simulink model "afe_dqctrl_param"  (R2026a)
settings: Solver=ode23tb  StopTime=param.sim.simlength  FixedStep=tc  MaxStep=param.glb_time.tc
values from neighbouring files (symbols this model uses):
  param = add_template_extras(param, options)    [init_model.m]
undefined symbols (not defined in the file or in its folder): magnitude
libraries: fl_lib x166, nesl_utility x91, igbt_simple_2th_lib x6, single_phase_transformer_lib x3, discrete_time_low_pass_filter x1, threephase_inductor_lib x1, dclink_for_two_levels x1, three_phase_pwm_modulator x1, three_phase_voltage_with_frt_emulator x1
(part 1 of 7)
settings Model: Creator=dbagn  LastModifiedBy=d.bagnara
settings SolverCC: NumberNewtonIterations=3.0  ZeroCrossControl=DisableAll  SolverResetMethod=Robust
settings SFSimCC: CustomCodeUndefinedFunction=ThrowError  DefaultCustomCodeDeterministicFunctions=All
settings SFSimCC: SimCustomHeaderCode=|
  | #include "rpi.h"
  | #include "rpi_simulink.h"
  | #include "bemf_obsv_load_est.h"
  | #include "bemf_obsv_load_est_simulink.h"
  | #include "dqpll_grid.h"
  | #include "dsmavgflt.h"
  | #include "bemf_obsv.h"
  | #include "bemf_obsv_simulink.h"
  | #include "mavgflt.h"
  | #include "mavgflt_simulink.h"
  | #include "mavgflts.h"
  | #include "mavgflts_simulink.h"
  | #include "sv_pwm_cm.h"
  | #include "dsmavgflt_simulink.h"
  | #include "linear_double_integrator_observer_simulink.h"
  | #include "sv_pwm_cm_simulink.h"
  | #include "dqvector_pi.h"
  | #include "dqpll_grid_simulink.h"
  | #include "first_harmonic_tracker.h"
  | #include "dqvector_pi_simulink.h"
  | #include "first_harmonic_tracker_simulink.h"
  | #include "dqpll_thyr.h"
  | #include "sv_pwm_simulink.h"
  | #include "sv_pwm.h"
  | #include "dqpll_thyr_simulink.h"
  | #include "linear_double_integrator_observer.h"
  | #include "math_f.h"
settings SFSimCC: SimUserSources=|
  | "rpi.c"
  | "rpi_simulink.c"
  | "mavgflt_simulink.c"
  | "mavgflt.c"
  | "mavgflts_simulink.c"
  | "mavgflts.c"
  | "dsmavgflt_simulink.c"
  | "dsmavgflt.c"
  | "bemf_obsv_simulink.c"
  | "bemf_obsv.c"
  | "bemf_obsv_load_est_simulink.c"
  | "bemf_obsv_load_est.c"
  | "dqvector_pi.c"
  | "dqvector_pi_simulink.c"
  | "sv_pwm_simulink.c"
  | "sv_pwm.c"
  | "first_harmonic_tracker_simulink.c"
  | "first_harmonic_tracker.c"
  | "dqpll_thyr_simulink.c"
  | "dqpll_thyr.c"
  | "dqpll_grid_simulink.c"
  | "dqpll_grid.c"
  | "linear_double_integrator_observer_simulink.c"
  | "linear_double_integrator_observer.c"
  | "sv_pwm_cm_simulink.c"
  | "sv_pwm_cm.c"
settings SFSimCC: SimUserIncludeDirs=|
  | include
  | src
settings SimscapeCC: SimscapeNominalValues="[{\"value\":\"1\",\"unit\":\"A\"},{\"value\":\"1\",\"unit\":\"bar\"},{\"value\":\"1\",\"unit\":\"cm^2\"},{\"value\":\"1\",\"unit\":\"cm^3/s\"},{\"value\":\"1\",\"unit\":\"kJ/kg\"},{\"value\":\"1\",\"unit\":\"kW\"},{\"value\":\"1\",\"unit\":\"l\"},{\"value\":\"1\",\"unit\":\"N\"},{\"value\":\"1\",\"unit\":\"N*m\"},{\"value\":\"1\",\"unit\":\"V\"}]"  SimscapeLogType=none  SimscapeLogDataHistory=5000.0

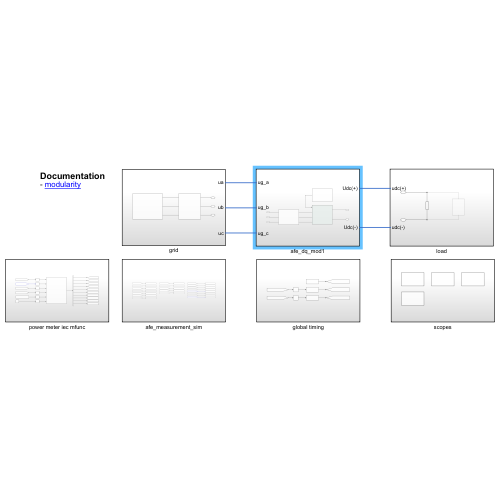
[thumbnail: Simulink's stored preview of the top-level diagram]
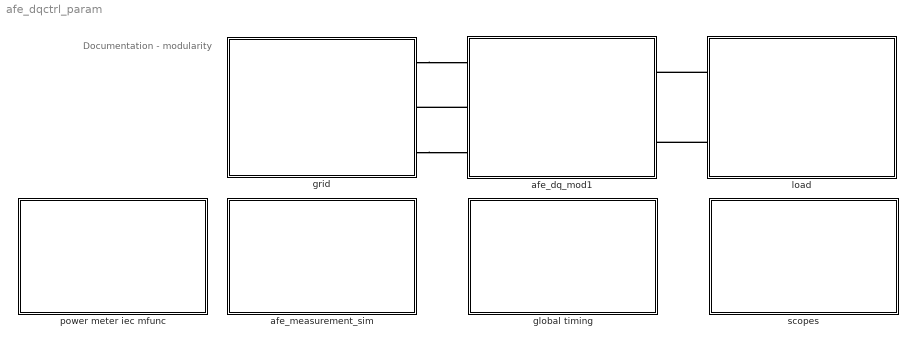
== system afe_dqctrl_param ==
  note: Documentation
      | - modularity
  afe_dq_mod1 : Subsystem
  afe_measurement_sim : Subsystem
  global timing : Subsystem
  grid : Subsystem
  load : Subsystem
  power meter iec mfunc : Subsystem
  scopes : Subsystem
  connections:
  grid/RConn1 -- afe_dq_mod1/LConn1
  grid/RConn3 -- afe_dq_mod1/LConn3
  afe_dq_mod1/LConn2 -- grid/RConn2
  load/LConn1 -- afe_dq_mod1/RConn1
  load/LConn2 -- afe_dq_mod1/RConn2

== system afe_dqctrl_param/afe_dq_mod1 ==
  AFE_control : Subsystem
  LCL_filter : Subsystem
  afe : Subsystem
  ug_a : PMIOPort  Side=Left
  ug_b : PMIOPort  Port=2  Side=Left
  ug_c : PMIOPort  Port=3  Side=Left
  Udc(+) : PMIOPort  Port=4  Side=Right
  Udc(-) : PMIOPort  Port=5  Side=Right
  wires:
  AFE_control/1(dabc_out) -> afe/1(dabc)
  connections:
  Udc(-)/RConn1 -- afe/RConn2
  Udc(+)/RConn1 -- afe/RConn1
  LCL_filter/LConn1 -- afe/LConn1
  LCL_filter/LConn2 -- afe/LConn2
  LCL_filter/LConn3 -- afe/LConn3
  ug_a/RConn1 -- LCL_filter/RConn1
  ug_b/RConn1 -- LCL_filter/RConn2
  ug_c/RConn1 -- LCL_filter/RConn3

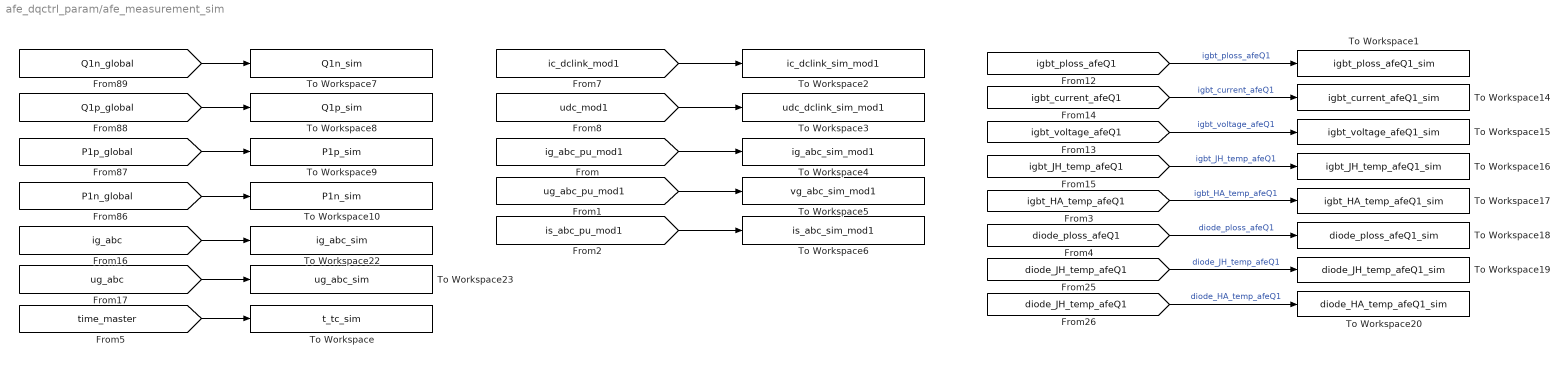
== system afe_dqctrl_param/afe_measurement_sim ==
  To Workspace : ToWorkspace  VariableName=t_tc_sim  SampleTime=param.glb_time.tc
      settings: MaxDataPoints=param.glb_time.Nc
  To Workspace1 : ToWorkspace  VariableName=igbt_ploss_afeQ1_sim  SampleTime=param.glb_time.tc
      settings: MaxDataPoints=param.glb_time.Nc
  To Workspace10 : ToWorkspace  VariableName=P1n_sim  SampleTime=param.glb_time.ts_afe
      settings: MaxDataPoints=param.glb_time.Ns_afe
  To Workspace14 : ToWorkspace  VariableName=igbt_current_afeQ1_sim  SampleTime=param.glb_time.tc
      settings: MaxDataPoints=param.glb_time.Nc
  To Workspace15 : ToWorkspace  VariableName=igbt_voltage_afeQ1_sim  SampleTime=param.glb_time.tc
      settings: MaxDataPoints=param.glb_time.Nc
  To Workspace16 : ToWorkspace  VariableName=igbt_JH_temp_afeQ1_sim  SampleTime=param.glb_time.tc
      settings: MaxDataPoints=param.glb_time.Nc
  To Workspace17 : ToWorkspace  VariableName=igbt_HA_temp_afeQ1_sim  SampleTime=param.glb_time.tc
      settings: MaxDataPoints=param.glb_time.Nc
  To Workspace18 : ToWorkspace  VariableName=diode_ploss_afeQ1_sim  SampleTime=param.glb_time.tc
      settings: MaxDataPoints=param.glb_time.Nc
  To Workspace19 : ToWorkspace  VariableName=diode_JH_temp_afeQ1_sim  SampleTime=param.glb_time.tc
      settings: MaxDataPoints=param.glb_time.Nc
  To Workspace2 : ToWorkspace  VariableName=ic_dclink_sim_mod1  SampleTime=param.glb_time.tc
      settings: MaxDataPoints=param.glb_time.Nc
  To Workspace20 : ToWorkspace  VariableName=diode_HA_temp_afeQ1_sim  SampleTime=param.glb_time.tc
      settings: MaxDataPoints=param.glb_time.Nc
  To Workspace22 : ToWorkspace  VariableName=ig_abc_sim  SampleTime=param.glb_time.tc
      settings: MaxDataPoints=param.glb_time.Nc
  To Workspace23 : ToWorkspace  VariableName=ug_abc_sim  SampleTime=param.glb_time.tc
      settings: MaxDataPoints=param.glb_time.Nc
  To Workspace3 : ToWorkspace  VariableName=udc_dclink_sim_mod1  SampleTime=param.glb_time.tc
      settings: MaxDataPoints=param.glb_time.Nc
  To Workspace4 : ToWorkspace  VariableName=ig_abc_sim_mod1  SampleTime=param.glb_time.tc
      settings: MaxDataPoints=param.glb_time.Nc
  To Workspace5 : ToWorkspace  VariableName=vg_abc_sim_mod1  SampleTime=param.glb_time.tc
      settings: MaxDataPoints=param.glb_time.Nc
  To Workspace6 : ToWorkspace  VariableName=is_abc_sim_mod1  SampleTime=param.glb_time.tc
      settings: MaxDataPoints=param.glb_time.Nc
  To Workspace7 : ToWorkspace  VariableName=Q1n_sim  SampleTime=param.glb_time.ts_afe
      settings: MaxDataPoints=param.glb_time.Ns_afe
  To Workspace8 : ToWorkspace  VariableName=Q1p_sim  SampleTime=param.glb_time.ts_afe
      settings: MaxDataPoints=param.glb_time.Ns_afe
  To Workspace9 : ToWorkspace  VariableName=P1p_sim  SampleTime=param.glb_time.ts_afe
      settings: MaxDataPoints=param.glb_time.Ns_afe
  wires:
  [time_master] -> To Workspace/1
  [Q1n_global] -> To Workspace7/1
  [Q1p_global] -> To Workspace8/1
  [P1p_global] -> To Workspace9/1
  [P1n_global] -> To Workspace10/1
  [ug_abc] -> To Workspace23/1
  [ig_abc] -> To Workspace22/1
  [ug_abc_pu_mod1] -> To Workspace5/1
  [ig_abc_pu_mod1] -> To Workspace4/1
  [udc_mod1] -> To Workspace3/1
  [ic_dclink_mod1] -> To Workspace2/1
  [is_abc_pu_mod1] -> To Workspace6/1
  [igbt_voltage_afeQ1] -> To Workspace15/1  "igbt_voltage_afeQ1"
  [igbt_HA_temp_afeQ1] -> To Workspace17/1  "igbt_HA_temp_afeQ1"
  [diode_ploss_afeQ1] -> To Workspace18/1  "diode_ploss_afeQ1"
  [diode_JH_temp_afeQ1] -> To Workspace19/1  "diode_JH_temp_afeQ1"
  [igbt_ploss_afeQ1] -> To Workspace1/1  "igbt_ploss_afeQ1"
  [diode_JH_temp_afeQ1] -> To Workspace20/1  "diode_HA_temp_afeQ1"
  [igbt_current_afeQ1] -> To Workspace14/1  "igbt_current_afeQ1"
  [igbt_JH_temp_afeQ1] -> To Workspace16/1  "igbt_JH_temp_afeQ1"

== system afe_dqctrl_param/global timing ==
  Unit Delay : UnitDelay  SampleTime=param.glb_time.tc
  Unit Delay1 : UnitDelay  SampleTime=param.glb_time.tc
  time_afe1 : Subsystem  mask{k=param.afe.behav.time_gain_module_1}
      mask prompts: k "Time Gain"
      mask Display:
      | disp('time-gen');
      | port_label('input', 1, 'crt');
      | port_label('output', 1, 'tout');
  time_afe3 : Subsystem  mask{k=1}
      mask prompts: k "Time Gain"
      mask Display:
      | disp('time-gen');
      | port_label('output', 1, 'tout');
  time_inv1 : Subsystem  mask{k=param.inv.behav.time_gain_module_2}
      mask prompts: k "Time Gain"
      mask Display:
      | disp('time-gen');
      | port_label('input', 1, 'crt');
      | port_label('output', 1, 'tout');
  tag scope: time_afe_module_1=global, time_inv_module_1=global, time_master=global
  wires:
  time_afe1/1(Out1) -> [time_afe_module_1]
  time_inv1/1(Out1) -> [time_inv_module_1]
  time_afe3/1(Out1) -> [time_master]
  [local_time_corr_afe1] -> Unit Delay/1
  Unit Delay/1 -> time_afe1/1(correction_time)
  [local_time_corr_inv1] -> Unit Delay1/1
  Unit Delay1/1 -> time_inv1/1(correction_time)

== system afe_dqctrl_param/grid ==
  grid_emulator : Subsystem
  threephase_vi_measures : Subsystem
  ua : PMIOPort  Side=Right
  ub : PMIOPort  Port=2  Side=Right
  uc : PMIOPort  Port=3  Side=Right
  connections:
  threephase_vi_measures/LConn3 -- grid_emulator/RConn3
  threephase_vi_measures/LConn1 -- grid_emulator/RConn1
  threephase_vi_measures/RConn2 -- ub/RConn1
  threephase_vi_measures/LConn2 -- grid_emulator/RConn2
  threephase_vi_measures/RConn1 -- ua/RConn1
  threephase_vi_measures/RConn3 -- uc/RConn1

== system afe_dqctrl_param/load ==
  load : fl_lib/Electrical/Electrical Elements/Resistor  R=1070^2/275e3 Ohm  i_specify=off  i_priority=None  i=0 A  i_nominal_specify=off  i_nominal_value=1  i_nominal_unit=A  v_specify=off  v_priority=None  v=0 V  v_nominal_specify=off  v_nominal_value=1  v_nominal_unit=V
  load_current_source : Subsystem  Commented=on
  udc(+) : PMIOPort  Side=Left
  udc(-) : PMIOPort  Port=2  Side=Left
  connections:
  load/RConn1 -- udc(-)/RConn1 -- load_current_source/RConn1
  udc(+)/RConn1 -- load_current_source/LConn1 -- load/LConn1

== system afe_dqctrl_param/power meter iec mfunc ==
  Bus Selector : BusSelector  OutputSignals=Q1p,Q1n,P1n,P1p,U1n,U1p,i_act_1n,i_react_1n,i_act_1p,i_react_1p
  Constant : Constant  Value=param.glb_time.ts_afe
  Step : Step  Time=0.025  InitialValue=1  FinalValue=0  SampleTime=0
  To Workspace1 : ToWorkspace  VariableName=i_react_1n  SampleTime=param.glb_time.ts_afe
      settings: MaxDataPoints=param.glb_time.Ns_afe
  To Workspace2 : ToWorkspace  VariableName=i_react_1p  SampleTime=param.glb_time.ts_afe
      settings: MaxDataPoints=param.glb_time.Ns_afe
  To Workspace3 : ToWorkspace  VariableName=i_act_1n  SampleTime=param.glb_time.ts_afe
      settings: MaxDataPoints=param.glb_time.Ns_afe
  To Workspace4 : ToWorkspace  VariableName=i_act_1p  SampleTime=param.glb_time.ts_afe
      settings: MaxDataPoints=param.glb_time.Ns_afe
  To Workspace5 : ToWorkspace  VariableName=u1p  SampleTime=param.glb_time.ts_afe
      settings: MaxDataPoints=param.glb_time.Ns_afe
  To Workspace6 : ToWorkspace  VariableName=u1n  SampleTime=param.glb_time.ts_afe
      settings: MaxDataPoints=param.glb_time.Ns_afe
  Zero-Order Hold{,1..5} (6 alike) : ZeroOrderHold  SampleTime=param.glb_time.ts_afe
  three_phase_power_meter_iec : MATLAB Function  TreatAsAtomicUnit=on  SystemSampleTime=param.glb_time.ts_afe
  tag scope: P1n_global=global, P1p_global=global, Q1n_global=global, Q1p_global=global
  wires:
  Bus Selector/6 -> To Workspace5/1  "<U1p>"
  Bus Selector/8 -> To Workspace1/1  "<i_react_1n>"
  Bus Selector/10 -> To Workspace2/1  "<i_react_1p>"
  Bus Selector/5 -> To Workspace6/1  "<U1n>"
  Bus Selector/4 -> [P1p_global]  "<P1p>"
  Bus Selector/2 -> [Q1n_global]  "<Q1n>"
  Bus Selector/1 -> [Q1p_global]  "<Q1p>"
  Bus Selector/7 -> To Workspace3/1  "<i_act_1n>"
  Bus Selector/9 -> To Workspace4/1  "<i_act_1p>"
  Bus Selector/3 -> [P1n_global]  "<P1n>"
  three_phase_power_meter_iec/1(m) -> Bus Selector/1
  Zero-Order Hold/1 -> three_phase_power_meter_iec/1(phase)
  Zero-Order Hold2/1 -> three_phase_power_meter_iec/3(i_abc)
  [gamma_grid_emulator] -> Zero-Order Hold/1
  Step/1 -> Zero-Order Hold5/1
  Zero-Order Hold3/1 -> three_phase_power_meter_iec/4(omega)
  Zero-Order Hold4/1 -> three_phase_power_meter_iec/5(ts)
  [ug_abc] -> Zero-Order Hold1/1
  Zero-Order Hold5/1 -> three_phase_power_meter_iec/6(enable_time)
  [ig_abc] -> Zero-Order Hold2/1
  [omega_grid_emulator] -> Zero-Order Hold3/1
  Constant/1 -> Zero-Order Hold4/1
  Zero-Order Hold1/1 -> three_phase_power_meter_iec/2(u_abc)

== system afe_dqctrl_param/scopes ==
  cable_effects : Subsystem
  grid_afe_side : Subsystem
  igbt_power_losses : Subsystem
  mosfet_power_losses : Subsystem  Commented=on

== system afe_dqctrl_param/afe_dq_mod1/AFE_control ==
  To Workspace : ToWorkspace  VariableName=afe_ctrl_data_output_mod1  SampleTime=param.glb_time.ts_afe
      settings: MaxDataPoints=param.glb_time.Ns_afe
  afe_control : Subsystem
  dabc_out : Outport
  tag scope: local_time_corr_afe1=global
  wires:
  [TRGO_afe_module_1] -> afe_control/Trigger
  [ug_abc_pu_mod1] -> afe_control/1(ug_abc_pu)
  [is_abc_pu_mod1] -> afe_control/4(is_abc_pu)
  [vdc_pu_afe_mod1] -> afe_control/2(udc_pu)
  afe_control/1(duvw) -> dabc_out/1
  [ig_abc_pu_mod1] -> afe_control/3(ig_abc_pu)
  [time_afe_module_1] -> afe_control/5(local_time)
  [time_master] -> afe_control/6(master_time)
  [gamma_grid_emulator] -> afe_control/7(grid_phase)
  afe_control/3(m_data) -> To Workspace/1
  afe_control/2(AFE1_local_time_corr) -> [local_time_corr_afe1]

== system afe_dqctrl_param/afe_dq_mod1/LCL_filter ==
  CFu1 : fl_lib/Electrical/Electrical Elements/Capacitor  c=param.afe.hw.CFu F  r=param.afe.hw.RCFu Ohm  g=0 1/Ohm  i_specify=off  i_priority=None  i=0 A  i_nominal_specify=off  i_nominal_value=1  i_nominal_unit=A  v_specify=off  v_priority=None  v=0 V  v_nominal_specify=off  v_nominal_value=1  v_nominal_unit=V  vc_specify=off  vc_priority=High  vc=0 V  vc_nominal_specify=off  vc_nominal_value=1  vc_nominal_unit=V
  CFu2 : fl_lib/Electrical/Electrical Elements/Capacitor  c=param.afe.hw.CFu F  r=param.afe.hw.RCFu Ohm  g=0 1/Ohm  i_specify=off  i_priority=None  i=0 A  i_nominal_specify=off  i_nominal_value=1  i_nominal_unit=A  v_specify=off  v_priority=None  v=0 V  v_nominal_specify=off  v_nominal_value=1  v_nominal_unit=V  vc_specify=off  vc_priority=High  vc=0 V  vc_nominal_specify=off  vc_nominal_value=1  vc_nominal_unit=V
  CFu3 : fl_lib/Electrical/Electrical Elements/Capacitor  c=param.afe.hw.CFu F  r=param.afe.hw.RCFu Ohm  g=0 1/Ohm  i_specify=off  i_priority=None  i=0 A  i_nominal_specify=off  i_nominal_value=1  i_nominal_unit=A  v_specify=off  v_priority=None  v=0 V  v_nominal_specify=off  v_nominal_value=1  v_nominal_unit=V  vc_specify=off  vc_priority=High  vc=0 V  vc_nominal_specify=off  vc_nominal_value=1  vc_nominal_unit=V
  Inductor : fl_lib/Electrical/Electrical Elements/Inductor  l=1e-6 H  r=0 Ohm  g=1e-9 1/Ohm  i_specify=on  i_priority=High  i=0 A  i_nominal_specify=off  i_nominal_value=1  i_nominal_unit=A  v_specify=off  v_priority=None  v=0 V  v_nominal_specify=off  v_nominal_value=1  v_nominal_unit=V  i_L_specify=off  i_L_priority=High  i_L=0 A  i_L_nominal_specify=off  i_L_nominal_value=1  i_L_nominal_unit=A
  Inductor1 : fl_lib/Electrical/Electrical Elements/Inductor  l=1e-6 H  r=0 Ohm  g=1e-9 1/Ohm  i_specify=on  i_priority=High  i=0 A  i_nominal_specify=off  i_nominal_value=1  i_nominal_unit=A  v_specify=off  v_priority=None  v=0 V  v_nominal_specify=off  v_nominal_value=1  v_nominal_unit=V  i_L_specify=off  i_L_priority=High  i_L=0 A  i_L_nominal_specify=off  i_L_nominal_value=1  i_L_nominal_unit=A
  Inductor2 : fl_lib/Electrical/Electrical Elements/Inductor  l=1e-6 H  r=0 Ohm  g=1e-9 1/Ohm  i_specify=on  i_priority=High  i=0 A  i_nominal_specify=off  i_nominal_value=1  i_nominal_unit=A  v_specify=off  v_priority=None  v=0 V  v_nominal_specify=off  v_nominal_value=1  v_nominal_unit=V  i_L_specify=off  i_L_priority=High  i_L=0 A  i_L_nominal_specify=off  i_L_nominal_value=1  i_L_nominal_unit=A
  threephase inductor : threephase_inductor_lib/threephase inductor  Lp=param.afe.hw.LFu H  L0=param.afe.hw.LFu_cm H  Rp=param.afe.hw.RLFu Ohm  R0=param.afe.hw.RLFu_cm Ohm  Lls=5e-6 H  uu_1_specify=off  uu_1_priority=None  uu_1=0 V  uu_1_nominal_specify=off  uu_1_nominal_value=1  uu_1_nominal_unit=V  uv_1_specify=off  uv_1_priority=None  uv_1=0 V  uv_1_nominal_specify=off  uv_1_nominal_value=1  uv_1_nominal_unit=V  uw_1_specify=off  uw_1_priority=None  uw_1=0 V  uw_1_nominal_specify=off  uw_1_nominal_value=1  uw_1_nominal_unit=V  uu_2_specify=off  uu_2_priority=None  uu_2=0 V  uu_2_nominal_specify=off  uu_2_nominal_value=1  uu_2_nominal_unit=V  uv_2_specify=off  uv_2_priority=None  uv_2=0 V  uv_2_nominal_specify=off  uv_2_nominal_value=1  uv_2_nominal_unit=V  uw_2_specify=off  uw_2_priority=None  uw_2=0 V  uw_2_nominal_specify=off  uw_2_nominal_value=1  uw_2_nominal_unit=V  iu_specify=off  iu_priority=High  iu=0 A  iu_nominal_specify=off  iu_nominal_value=1  iu_nominal_unit=A  iv_specify=off  iv_priority=High  iv=0 A  iv_nominal_specify=off  iv_nominal_value=1  iv_nominal_unit=A  iw_specify=off  iw_priority=High  iw=0 A  iw_nominal_specify=off  iw_nominal_value=1  iw_nominal_unit=A
  threephase_vi_measures_stack : Subsystem
  threephase_vi_measures_stack1 : Subsystem
  us_a : PMIOPort  Side=Left
  ug_a : PMIOPort  Port=2  Side=Right
  us_b : PMIOPort  Port=3  Side=Left
  ug_b : PMIOPort  Port=4  Side=Right
  us_c : PMIOPort  Port=5  Side=Left
  ug_c : PMIOPort  Port=6  Side=Right
  connections:
  CFu1/RConn1 -- CFu3/RConn1 -- CFu2/RConn1
  Inductor/RConn1 -- threephase_vi_measures_stack1/LConn1 -- CFu1/LConn1
  Inductor2/RConn1 -- CFu3/LConn1 -- threephase_vi_measures_stack1/LConn3
  Inductor1/RConn1 -- CFu2/LConn1 -- threephase_vi_measures_stack1/LConn2
  threephase_vi_measures_stack/LConn1 -- us_a/RConn1
  threephase_vi_measures_stack/LConn2 -- us_b/RConn1
  threephase_vi_measures_stack/LConn3 -- us_c/RConn1
  threephase_vi_measures_stack/RConn1 -- threephase inductor/LConn1
  threephase_vi_measures_stack/RConn2 -- threephase inductor/LConn2
  threephase_vi_measures_stack/RConn3 -- threephase inductor/LConn3
  threephase inductor/RConn1 -- Inductor/LConn1
  Inductor1/LConn1 -- threephase inductor/RConn2
  Inductor2/LConn1 -- threephase inductor/RConn3
  ug_a/RConn1 -- threephase_vi_measures_stack1/RConn1
  ug_b/RConn1 -- threephase_vi_measures_stack1/RConn2
  ug_c/RConn1 -- threephase_vi_measures_stack1/RConn3

== system afe_dqctrl_param/afe_dq_mod1/afe ==
  dabc : Inport
  Bus Selector : BusSelector  OutputSignals=vdc_pu
  Bus Selector1 : BusSelector  OutputSignals=udc,udc_p_gnd,udc_centertap_gnd,udc_n_gnd  OutputAsBus=on
  Bus Selector2 : BusSelector  OutputSignals=udc
  Bus Selector3 : BusSelector  OutputSignals=Cdc1_current
  dclink1 : dclink_for_two_levels/dclink  Cdc=param.afe.hw.CFi  Rudc_measure=1e6  Vdc_scale=param.afe.hw.udc_nom
  sv_pwm : Subsystem
  three_phase_inverter_with_igbt_simple_2th : Subsystem
  us_a : PMIOPort  Side=Left
  us_b : PMIOPort  Port=2  Side=Left
  us_c : PMIOPort  Port=3  Side=Left
  Udc(+) : PMIOPort  Port=4  Side=Right
  Udc(-) : PMIOPort  Port=5  Side=Right
  tag scope: all_voltages_about_dclink=global, ic_dclink_mod1=global, udc_mod1=global, vdc_pu_afe_mod1=global, vdc_pu_inv_mod1=global
  wires:
  dabc/1 -> sv_pwm/1(duties_uvw)
  sv_pwm/1(gate_cmds) -> three_phase_inverter_with_igbt_simple_2th/1(gate_commands)
  dclink1/1 -> Bus Selector1/1, Bus Selector2/1, Bus Selector3/1, Bus Selector/1
  Bus Selector1/1 -> [all_voltages_about_dclink]
  Bus Selector/1 -> [vdc_pu_afe_mod1], [vdc_pu_inv_mod1]  "<vdc_pu>"
  Bus Selector2/1 -> [udc_mod1]  "<udc>"
  Bus Selector3/1 -> [ic_dclink_mod1]  "<Cdc1_current>"
  connections:
  three_phase_inverter_with_igbt_simple_2th/RConn2 -- us_b/RConn1
  dclink1/RConn1 -- Udc(+)/RConn1
  dclink1/RConn2 -- Udc(-)/RConn1
  three_phase_inverter_with_igbt_simple_2th/RConn1 -- us_a/RConn1
  three_phase_inverter_with_igbt_simple_2th/RConn3 -- us_c/RConn1
  dclink1/LConn2 -- three_phase_inverter_with_igbt_simple_2th/LConn2
  dclink1/LConn1 -- three_phase_inverter_with_igbt_simple_2th/LConn1

== system afe_dqctrl_param/global timing/time_afe1 ==
  correction_time : Inport
  Constant : Constant
  Gain : Gain  Gain=k
  Product : Product
  Sum : Sum  Inputs=|++
  time_1 : Clock
  Out1 : Outport
  wires:
  time_1/1 -> Gain/1
  Gain/1 -> Product/1
  Product/1 -> Out1/1
  correction_time/1 -> Sum/1
  Sum/1 -> Product/2
  Constant/1 -> Sum/2

== system afe_dqctrl_param/global timing/time_afe3 ==
  Gain : Gain  Gain=k
  time_1 : Clock
  Out1 : Outport
  wires:
  Gain/1 -> Out1/1
  time_1/1 -> Gain/1

== system afe_dqctrl_param/global timing/time_inv1 ==
  correction_time : Inport
  Constant : Constant
  Gain : Gain  Gain=k
  Product : Product
  Sum : Sum  Inputs=|++
  time_1 : Clock
  Out1 : Outport
  wires:
  time_1/1 -> Gain/1
  Gain/1 -> Product/1
  Product/1 -> Out1/1
  correction_time/1 -> Sum/1
  Constant/1 -> Sum/2
  Sum/1 -> Product/2

== system afe_dqctrl_param/grid/grid_emulator ==
  3ph_Dyg : Subsystem
  Bus Selector : BusSelector  OutputSignals=ua_grid_emu,ub_grid_emu,uc_grid_emu
  Bus Selector1 : BusSelector  OutputSignals=gamma_grid_emulator,omega_grid_emulator
  Controlled Voltage Source : fl_lib/Electrical/Electrical Sources/Controlled Voltage Source
  Controlled Voltage Source1 : fl_lib/Electrical/Electrical Sources/Controlled Voltage Source
  Controlled Voltage Source2 : fl_lib/Electrical/Electrical Sources/Controlled Voltage Source
  Electrical Reference : fl_lib/Electrical/Electrical Elements/Electrical Reference
  Simulink-PS Converter : nesl_utility/Simulink-PS Converter  PhysicalDomain=network_engine_domain  SubClassName=ps_input  LeftPortType=input  RightPortType=output  PseudoPeriodic=off  Frequencies=[]  NoiseDistribution=none  NoiseParameters=[]  Unit=V  AffineConversion=on  FilteringAndDerivatives=provide  SimscapeFilterOrder=1  InputFilterTimeConstant=0.001  UdotUserProvided=0
  Simulink-PS Converter1 : nesl_utility/Simulink-PS Converter  PhysicalDomain=network_engine_domain  SubClassName=ps_input  LeftPortType=input  RightPortType=output  PseudoPeriodic=off  Frequencies=[]  NoiseDistribution=none  NoiseParameters=[]  Unit=V  AffineConversion=on  FilteringAndDerivatives=provide  SimscapeFilterOrder=1  InputFilterTimeConstant=0.001  UdotUserProvided=0
  Simulink-PS Converter2 : nesl_utility/Simulink-PS Converter  PhysicalDomain=network_engine_domain  SubClassName=ps_input  LeftPortType=input  RightPortType=output  PseudoPeriodic=off  Frequencies=[]  NoiseDistribution=none  NoiseParameters=[]  Unit=V  AffineConversion=on  FilteringAndDerivatives=provide  SimscapeFilterOrder=1  InputFilterTimeConstant=0.001  UdotUserProvided=0
  Solver Configuration : nesl_utility/Solver Configuration  PhysicalDomain=network_engine_domain  SubClassName=solver  LeftPortType=input  RightPortType=generic  Tones=[]  Harmonics=[]  SimulateNoise=off  Profile=off  UseLocalSampling=off  EnableSwitchedLinearOptims=on  FrequencyDomain=off  UseCCode=off  RelTol=0.001  AbsTol=0.001  MinStep=1e-09  ToWorkspace=off  RevertToSquareIcSolve=off  NumHomotopyIterations=100  PhasorMode=off  PhasorModeNumHarmonics=1  ConsistencySolver=NEWTON_FTOL  CanonicalOrdering=UNORDERED  OptimizeIntermediates=UNOPTIMIZED  IndexReductionMethod=DerivativeReplacement  DoDC=on  ResidualTolerance=1e-3  ConsistencyTolSource=GLOBAL  ConsistencyAbsTol=0.001  ConsistencyRelTol=0.001  ConsistencyTolFactor=0.001  UseLocalSolver=on  LocalSolverChoice=NE_BACKWARD_EULER_ADVANCER  ResolveIndetEquations=on  FunctionEvalNumThread=1  LocalSolverSampleTime=param.glb_time.tc  DoFixedCost=on  MaxNonlinIter=param.sim.nonlinear_iterations  MaxModeIter=2  ComputeImpulses=off  ImpulseIterations=2  LinearAlgebra=auto  LinearAlgebraNumThread=0  EquationFormulation=NE_TIME_EF  DelaysMemoryBudget=1024  AutomaticFiltering=on  FilteringTimeConstant=0.001  PartitionStorageMethod=AS_NEEDED  PartitionMemoryBudget=1024  PartitionMethod=ROBUST  MultibodyUseLocalSolver=off  MultibodyLocalSolverChoice=ODE1  MultibodyLocalSolverSampleTime=0.001
  three_phase_voltage_source_with_frt_emulator : three_phase_voltage_with_frt_emulator/three_phase_voltage_source_with_frt_emulator  nominal_frequency_m=param.grid.emu.fgrid_nom  nominal_voltage_m=param.grid.emu.us_primary_nom  Vemu_ref_norm_m=param.grid.emu.Vemu_ref_norm  vp_xi_pu_m=param.grid.emu.up_xi_pu_ref  vp_eta_pu_m=param.grid.emu.up_eta_pu_ref  vn_xi_pu_m=param.grid.emu.un_xi_pu_ref  vn_eta_pu_m=param.grid.emu.un_eta_pu_ref  Am=param.ctrl.filters.afe.SOF_50Hz.ss_c.A  Bm=param.ctrl.filters.afe.SOF_50Hz.ss_c.B  Cm=param.ctrl.filters.afe.SOF_50Hz.ss_c.C  enable_frt_1_m=param.frt.data.enable_frt_1  enable_frt_2_m=param.frt.data.enable_frt_2  start_time_LVRT_m=param.frt.data.start_time_LVRT  end_time_LVRT_m=param.frt.data.end_time_LVRT  deepPOSxi_m=param.frt.data.deepPOSxi  deepPOSeta_m=param.frt.data.deepPOSeta  deepNEGxi_m=param.frt.data.deepNEGxi  deepNEGeta_m=param.frt.data.deepNEGeta  Amplitude_U_m=param.frt.data.Amplitude_U  Amplitude_V_m=param.frt.data.Amplitude_V  Amplitude_W_m=param.frt.data.Amplitude_W  t_ramp_m=param.frt.data.t_ramp  Phase_shift_m=param.frt.data.Phase_shift
  threephase_vi_measures : Subsystem
  u1 : PMIOPort  Side=Right
  u2 : PMIOPort  Port=2  Side=Right
  u3 : PMIOPort  Port=3  Side=Right
  tag scope: gamma_grid_emulator=global, omega_grid_emulator=global
  wires:
  Bus Selector1/2 -> [omega_grid_emulator]  "<omega_grid_emulator>"
  Bus Selector1/1 -> [gamma_grid_emulator]  "<gamma_grid_emulator>"
  Bus Selector/2 -> Simulink-PS Converter1/1  "<ub_grid_emu>"
  Bus Selector/3 -> Simulink-PS Converter2/1  "<uc_grid_emu>"
  three_phase_voltage_source_with_frt_emulator/1 -> Bus Selector1/1, Bus Selector/1
  Bus Selector/1 -> Simulink-PS Converter/1  "<ua_grid_emu>"
  connections:
  Simulink-PS Converter/RConn1 -- Controlled Voltage Source/RConn1
  Simulink-PS Converter1/RConn1 -- Controlled Voltage Source1/RConn1
  Simulink-PS Converter2/RConn1 -- Controlled Voltage Source2/RConn1
  Electrical Reference/LConn1 -- Controlled Voltage Source/RConn2 -- Controlled Voltage Source1/RConn2 -- Controlled Voltage Source2/RConn2 -- Solver Configuration/RConn1
  3ph_Dyg/RConn1 -- u1/RConn1
  3ph_Dyg/RConn2 -- u2/RConn1
  3ph_Dyg/RConn3 -- u3/RConn1
  3ph_Dyg/LConn1 -- threephase_vi_measures/RConn1
  3ph_Dyg/LConn2 -- threephase_vi_measures/RConn2
  3ph_Dyg/LConn3 -- threephase_vi_measures/RConn3
  Controlled Voltage Source/LConn1 -- threephase_vi_measures/LConn1
  Controlled Voltage Source1/LConn1 -- threephase_vi_measures/LConn2
  Controlled Voltage Source2/LConn1 -- threephase_vi_measures/LConn3

== system afe_dqctrl_param/grid/threephase_vi_measures ==
  Bus Creator : BusCreator  Inputs=6
  Current Sensor : fl_lib/Electrical/Electrical Sensors/Current Sensor
  Current Sensor1 : fl_lib/Electrical/Electrical Sensors/Current Sensor
  Current Sensor2 : fl_lib/Electrical/Electrical Sensors/Current Sensor
  Electrical Reference1 : fl_lib/Electrical/Electrical Elements/Electrical Reference
  Selector : Selector  InputPortWidth=6  IndexOptions=Index vector (dialog)  Indices=[1 2 3]  OutputSizes=1
  Selector1 : Selector  InputPortWidth=6  IndexOptions=Index vector (dialog)  Indices=[4 5 6]  OutputSizes=1
  Voltage Sensor : fl_lib/Electrical/Electrical Sensors/Voltage Sensor
  Voltage Sensor1 : fl_lib/Electrical/Electrical Sensors/Voltage Sensor
  Voltage Sensor2 : fl_lib/Electrical/Electrical Sensors/Voltage Sensor
  ia_grid : nesl_utility/PS-Simulink Converter  PhysicalDomain=network_engine_domain  SubClassName=ps_output  LeftPortType=input  RightPortType=output  PseudoPeriodic=off  Frequencies=[]  VectorFormat=1-D array  Unit=A  AffineConversion=off
  ib_grid : nesl_utility/PS-Simulink Converter  PhysicalDomain=network_engine_domain  SubClassName=ps_output  LeftPortType=input  RightPortType=output  PseudoPeriodic=off  Frequencies=[]  VectorFormat=1-D array  Unit=A  AffineConversion=off
  ic_grid : nesl_utility/PS-Simulink Converter  PhysicalDomain=network_engine_domain  SubClassName=ps_output  LeftPortType=input  RightPortType=output  PseudoPeriodic=off  Frequencies=[]  VectorFormat=1-D array  Unit=A  AffineConversion=off
  ig_abc/ug_abc : Scope  NumInputPorts=2
      settings: SampleTime=param.glb_time.tc  ActiveDisplayYMinimum=-728.92703752654245  ActiveDisplayYMaximum=734.90808013997  DataLoggingVariableName=ScopeData2
  ua_grid : nesl_utility/PS-Simulink Converter  PhysicalDomain=network_engine_domain  SubClassName=ps_output  LeftPortType=input  RightPortType=output  PseudoPeriodic=off  Frequencies=[]  VectorFormat=1-D array  Unit=V  AffineConversion=off
  ub_grid : nesl_utility/PS-Simulink Converter  PhysicalDomain=network_engine_domain  SubClassName=ps_output  LeftPortType=input  RightPortType=output  PseudoPeriodic=off  Frequencies=[]  VectorFormat=1-D array  Unit=V  AffineConversion=off
  uc_grid : nesl_utility/PS-Simulink Converter  PhysicalDomain=network_engine_domain  SubClassName=ps_output  LeftPortType=input  RightPortType=output  PseudoPeriodic=off  Frequencies=[]  VectorFormat=1-D array  Unit=V  AffineConversion=off
  Ua : PMIOPort  Side=Left
  ua : PMIOPort  Port=2  Side=Right
  Ub : PMIOPort  Port=3  Side=Left
  ub : PMIOPort  Port=4  Side=Right
  Uc : PMIOPort  Port=5  Side=Left
  uc : PMIOPort  Port=6  Side=Right
  tag scope: ig_abc=global, ug_abc=global
  wires:
  Bus Creator/1 -> Selector1/1, Selector/1  "vi_data"
  Selector/1 -> [ug_abc]
  ib_grid/1 -> Bus Creator/5  "ib"
  ia_grid/1 -> Bus Creator/4  "ia"
  ic_grid/1 -> Bus Creator/6  "ic"
  ua_grid/1 -> Bus Creator/1  "ua"
  ub_grid/1 -> Bus Creator/2  "ub"
  uc_grid/1 -> Bus Creator/3  "uc"
  Selector1/1 -> [ig_abc]
  [ug_abc] -> ig_abc/ug_abc/2  "ug_abc(line)"
  [ig_abc] -> ig_abc/ug_abc/1  "ig_abc(line)"
  connections:
  Current Sensor1/LConn1 -- Ub/RConn1 -- Voltage Sensor1/LConn1
  Electrical Reference1/LConn1 -- Voltage Sensor/RConn2 -- Voltage Sensor2/RConn2 -- Voltage Sensor1/RConn2
  Voltage Sensor/RConn1 -- ua_grid/LConn1
  Current Sensor/RConn2 -- ua/RConn1
  Voltage Sensor1/RConn1 -- ub_grid/LConn1
  Voltage Sensor2/LConn1 -- Current Sensor2/LConn1 -- Uc/RConn1
  Current Sensor/LConn1 -- Ua/RConn1 -- Voltage Sensor/LConn1
  Current Sensor1/RConn2 -- ub/RConn1
  Voltage Sensor2/RConn1 -- uc_grid/LConn1
  ib_grid/LConn1 -- Current Sensor1/RConn1
  ia_grid/LConn1 -- Current Sensor/RConn1
  ic_grid/LConn1 -- Current Sensor2/RConn1
  Current Sensor2/RConn2 -- uc/RConn1

== system afe_dqctrl_param/load/load_current_source ==
  PS Ramp : fl_lib/Physical Signals/Sources/PS Ramp  slope=4*275e3/1070 1/s  start_time=0 s  initial_output=0  ZeroCross=true
  PS Saturation : fl_lib/Physical Signals/Nonlinear Operators/PS Saturation  upper_limit=275e3/1070  lower_limit=-275e3/1070  ZeroCross=true
  load_current : fl_lib/Electrical/Electrical Sources/Controlled Current Source
  udc(+) : PMIOPort  Side=Left
  udc(-) : PMIOPort  Port=2  Side=Right
  connections:
  PS Ramp/RConn1 -- PS Saturation/LConn1
  PS Saturation/RConn1 -- load_current/RConn1
  udc(+)/RConn1 -- load_current/LConn1
  udc(-)/RConn1 -- load_current/RConn2

== system afe_dqctrl_param/scopes/cable_effects ==
  cable_effects : Scope  NumInputPorts=3
      settings: SampleTime=param.glb_time.tc  ActiveDisplayYMinimum=-7.1054273576010019E-14  ActiveDisplayYMaximum=7.1054273576010019E-14  DataLoggingVariableName=ScopeData35
  wires:
  [udc_pgnd] -> cable_effects/2
  [udc_ngnd] -> cable_effects/3
  [is_uvw_cm_mod1] -> cable_effects/1

== system afe_dqctrl_param/scopes/grid_afe_side ==
  Gain7 : Gain  Gain=param.afe.hw.ibez
  Gain8 : Gain  Gain=param.afe.hw.ubez
  Gain9 : Gain  Gain=param.afe.hw.ibez
  IEC_power_meter : Scope  NumInputPorts=4
      settings: ActiveDisplayString=4  ActiveDisplayYMinimum=-14783.360577936935  ActiveDisplayYMaximum=36549.01356956378  DataLoggingVariableName=ScopeData14
  i_line_abc/u_line_abc : Scope  NumInputPorts=2
      settings: SampleTime=param.glb_time.tc  ActiveDisplayYMinimum=-709.7301057575155  ActiveDisplayYMaximum=602.93232016103525  DataLoggingVariableName=ScopeData20
  idc/udc : Scope  NumInputPorts=2
      settings: SampleTime=param.glb_time.tc  ActiveDisplayYMinimum=-239.04322132962466  ActiveDisplayYMaximum=376.33870683328587  DataLoggingVariableName=ScopeData23
  ig_abc/ug_abc _mod1 : Scope  NumInputPorts=2
      settings: SampleTime=param.glb_time.tc  ActiveDisplayYMinimum=-1.1327683435596978  ActiveDisplayYMaximum=1.1407252992037524  DataLoggingVariableName=ScopeData22
  is_abc/us_abc _mod1 : Scope  NumInputPorts=3
      settings: SampleTime=param.glb_time.tc  ActiveDisplayYMinimum=306.0050369827876  ActiveDisplayYMaximum=344.53748899224172  DataLoggingVariableName=ScopeData21
  udc voltages : Scope  NumInputPorts=2
      settings: SampleTime=param.glb_time.tc  ActiveDisplayYMinimum=-0.15734078977800958  ActiveDisplayYMaximum=1.4160671074190738  DataLoggingVariableName=ScopeData24
  wires:
  [udc_mod1] -> idc/udc/2  "udc_dclink_mod1"
  [ug_abc_pu_mod1] -> ig_abc/ug_abc _mod1/2  "ug_abc_mod1"
  Gain8/1 -> is_abc/us_abc _mod1/2  "vs_abc_mod1"
  [ic_dclink_mod1] -> idc/udc/1  "ic_dclink_mod1"
  [is_abc_pu_mod1] -> Gain7/1
  [Q1p_global] -> IEC_power_meter/2  "Q1p_global"
  [all_voltages_about_dclink] -> udc voltages/2  "all_voltages_about_dclink"
  Gain7/1 -> is_abc/us_abc _mod1/1  "is_abc_mod1"
  [iz_afe_pu_mod1] -> Gain9/1
  [i_abc_line] -> i_line_abc/u_line_abc/1  "i_abc_line"
  [u_abc_line] -> i_line_abc/u_line_abc/2  "u_abc_line"
  [P1n_global] -> IEC_power_meter/4  "P1n_global"
  [ig_abc_pu_mod1] -> ig_abc/ug_abc _mod1/1  "ig_abc_mod1"
  [vs_abc_pu_mod1] -> Gain8/1
  [vdc_pu_afe_mod1] -> udc voltages/1  "udc"
  Gain9/1 -> is_abc/us_abc _mod1/3  "iz_afe_mod1"
  [Q1n_global] -> IEC_power_meter/1  "Q1n_global"
  [P1p_global] -> IEC_power_meter/3  "P1p_global"

== system afe_dqctrl_param/scopes/igbt_power_losses ==
  Bus Creator1 : BusCreator  Inputs=2
  Bus Creator11 : BusCreator  Inputs=2
  Bus Creator6 : BusCreator  Inputs=2
  diode power losses AFE Q1 : Scope  NumInputPorts=3
      settings: SampleTime=param.glb_time.tc  ActiveDisplayYMinimum=-43.518404437168776  ActiveDisplayYMaximum=391.66563993451905  DataLoggingVariableName=ScopeData32
  igbt power losses AFE Q1 : Scope  NumInputPorts=4
      settings: SampleTime=param.glb_time.tc  ActiveDisplayYMinimum=-49.116010955029296  ActiveDisplayYMaximum=442.04409859526379  DataLoggingVariableName=ScopeData15
  igbt power losses AFE Q2 : Scope  NumInputPorts=4
      settings: SampleTime=param.glb_time.tc  ActiveDisplayYMinimum=-40.548011363861626  ActiveDisplayYMaximum=364.9321022747547  DataLoggingVariableName=ScopeData26
  wires:
  [igbt_ploss_afeQ1] -> igbt power losses AFE Q1/1  "igbt_ploss_afeQ1"
  [igbt_current_afeQ2] -> igbt power losses AFE Q2/2  "igbt_current_afeQ2"
  [igbt_ploss_afeQ2] -> igbt power losses AFE Q2/1  "igbt_ploss_afeQ2"
  [igbt_JH_temp_afeQ1] -> Bus Creator1/1  "igbt_JH_temp_afeQ1"
  [diode_JH_temp_afeQ1] -> Bus Creator11/1  "diode_JH_temp_afeQ1"
  [igbt_JH_temp_afeQ2] -> Bus Creator6/1  "igbt_JH_temp_afeQ2"
  Bus Creator11/1 -> diode power losses AFE Q1/3
  [igbt_HA_temp_afeQ2] -> Bus Creator6/2  "igbt_HA_temp_afeQ2"
  [diode_HA_temp_afeQ1] -> Bus Creator11/2  "diode_HA_temp_afeQ1"
  Bus Creator1/1 -> igbt power losses AFE Q1/4
  Bus Creator6/1 -> igbt power losses AFE Q2/4
  [igbt_voltage_afeQ1] -> igbt power losses AFE Q1/3  "igbt_voltage_afeQ1"
  [igbt_current_afeQ1] -> igbt power losses AFE Q1/2  "igbt_current_afeQ1"
  [igbt_HA_temp_afeQ1] -> Bus Creator1/2  "igbt_HA_temp_afeQ1"
  [diode_ploss_afeQ1] -> diode power losses AFE Q1/2  "diode_ploss_afeQ1"
  [igbt_voltage_afeQ2] -> igbt power losses AFE Q2/3  "igbt_voltage_afeQ2"
  [diode_current_afeQ1] -> diode power losses AFE Q1/1  "diode_current_afeQ1"

== system afe_dqctrl_param/scopes/mosfet_power_losses ==
  Bus Creator8 : BusCreator  Inputs=2
  Bus Creator9 : BusCreator  Inputs=2
  mosfet power losses INV Q1 : Scope  NumInputPorts=4
      settings: SampleTime=param.glb_time.tc  ActiveDisplayYMinimum=-52.647210306071649  ActiveDisplayYMaximum=473.81757031333393  DataLoggingVariableName=ScopeData28
  mosfet power losses INV Q2 : Scope  NumInputPorts=4
      settings: SampleTime=param.glb_time.tc  ActiveDisplayYMinimum=-60.051099059926763  ActiveDisplayYMaximum=540.45256909803  DataLoggingVariableName=ScopeData29
  wires:
  [mosfet_current_invQ2] -> mosfet power losses INV Q2/3  "mosfet_current_invQ2"
  [mosfet_voltage_invQ1] -> mosfet power losses INV Q1/2  "mosfet_voltage_invQ1"
  [mosfet_HA_temp_invQ2] -> Bus Creator9/2  "mosfet_HA_temp_invQ2"
  [mosfet_JH_temp_invQ2] -> Bus Creator9/1  "mosfet_JH_temp_invQ2"
  [mosfet_ploss_invQ1] -> mosfet power losses INV Q1/1  "mosfet_ploss_invQ1"
  [mosfet_HA_temp_invQ1] -> Bus Creator8/2  "mosfet_HA_temp_invQ1"
  [mosfet_current_invQ1] -> mosfet power losses INV Q1/3  "mosfet_current_invQ1"
  Bus Creator8/1 -> mosfet power losses INV Q1/4
  [mosfet_voltage_invQ2] -> mosfet power losses INV Q2/2  "mosfet_voltage_invQ2"
  [mosfet_ploss_invQ2] -> mosfet power losses INV Q2/1  "mosfet_ploss_invQ2"
  Bus Creator9/1 -> mosfet power losses INV Q2/4
  [mosfet_JH_temp_invQ1] -> Bus Creator8/1  "mosfet_JH_temp_invQ1"

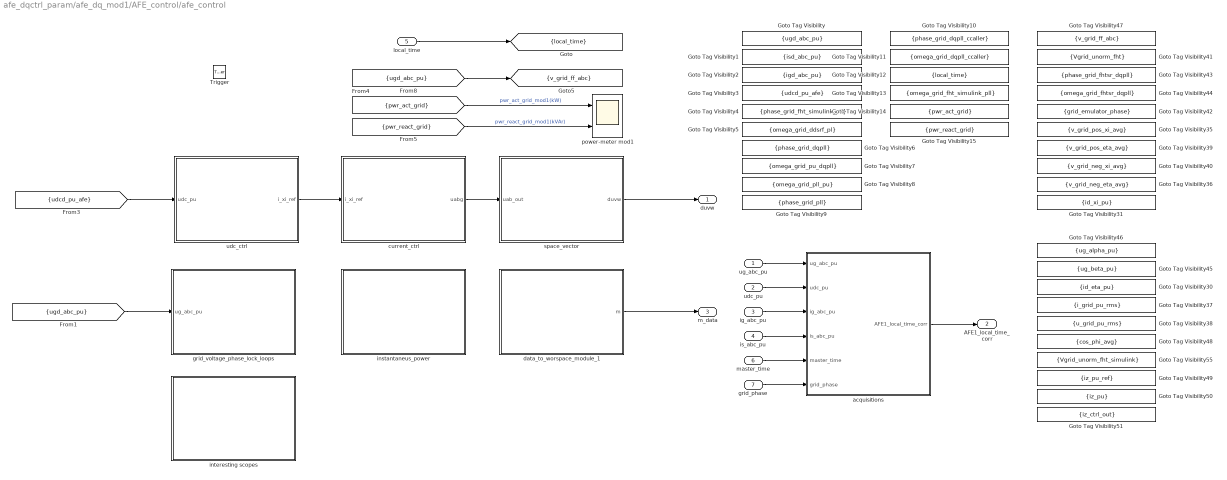
== system afe_dqctrl_param/afe_dq_mod1/AFE_control/afe_control ==
  ug_abc_pu : Inport
  udc_pu : Inport  Port=2
  ig_abc_pu : Inport  Port=3
  is_abc_pu : Inport  Port=4
  local_time : Inport  Port=5
  master_time : Inport  Port=6
  grid_phase : Inport  Port=7
  Trigger : TriggerPort  VariantControl=(inherit)  PortDimensions=1
  Goto Tag Visibility : GotoTagVisibility  GotoTag=ugd_abc_pu
  Goto Tag Visibility1 : GotoTagVisibility  GotoTag=isd_abc_pu
  Goto Tag Visibility10 : GotoTagVisibility  GotoTag=phase_grid_dqpll_ccaller
  Goto Tag Visibility11 : GotoTagVisibility  GotoTag=omega_grid_dqpll_ccaller
  Goto Tag Visibility12 : GotoTagVisibility  GotoTag=local_time
  Goto Tag Visibility13 : GotoTagVisibility  GotoTag=omega_grid_fht_simulink_pll
  Goto Tag Visibility14 : GotoTagVisibility  GotoTag=pwr_act_grid
  Goto Tag Visibility15 : GotoTagVisibility  GotoTag=pwr_react_grid
  Goto Tag Visibility2 : GotoTagVisibility  GotoTag=igd_abc_pu
  Goto Tag Visibility3 : GotoTagVisibility  GotoTag=udcd_pu_afe
  Goto Tag Visibility30 : GotoTagVisibility  GotoTag=id_eta_pu
  Goto Tag Visibility31 : GotoTagVisibility  GotoTag=id_xi_pu
  Goto Tag Visibility35 : GotoTagVisibility  GotoTag=v_grid_pos_xi_avg
  Goto Tag Visibility36 : GotoTagVisibility  GotoTag=v_grid_neg_eta_avg
  Goto Tag Visibility37 : GotoTagVisibility  GotoTag=i_grid_pu_rms
  Goto Tag Visibility38 : GotoTagVisibility  GotoTag=u_grid_pu_rms
  Goto Tag Visibility39 : GotoTagVisibility  GotoTag=v_grid_pos_eta_avg
  Goto Tag Visibility4 : GotoTagVisibility  GotoTag=phase_grid_fht_simulink_pll
  Goto Tag Visibility40 : GotoTagVisibility  GotoTag=v_grid_neg_xi_avg
  Goto Tag Visibility41 : GotoTagVisibility  GotoTag=Vgrid_unorm_fht
  Goto Tag Visibility42 : GotoTagVisibility  GotoTag=grid_emulator_phase
  Goto Tag Visibility43 : GotoTagVisibility  GotoTag=phase_grid_fhtsr_dqpll
  Goto Tag Visibility44 : GotoTagVisibility  GotoTag=omega_grid_fhtsr_dqpll
  Goto Tag Visibility45 : GotoTagVisibility  GotoTag=ug_beta_pu
  Goto Tag Visibility46 : GotoTagVisibility  GotoTag=ug_alpha_pu
  Goto Tag Visibility47 : GotoTagVisibility  GotoTag=v_grid_ff_abc
  Goto Tag Visibility48 : GotoTagVisibility  GotoTag=cos_phi_avg
  Goto Tag Visibility49 : GotoTagVisibility  GotoTag=iz_pu_ref
  Goto Tag Visibility5 : GotoTagVisibility  GotoTag=omega_grid_ddsrf_pl
  Goto Tag Visibility50 : GotoTagVisibility  GotoTag=iz_pu
  Goto Tag Visibility51 : GotoTagVisibility  GotoTag=iz_ctrl_out
  Goto Tag Visibility55 : GotoTagVisibility  GotoTag=Vgrid_unorm_fht_simulink
  Goto Tag Visibility6 : GotoTagVisibility  GotoTag=phase_grid_dqpll
  Goto Tag Visibility7 : GotoTagVisibility  GotoTag=omega_grid_pu_dqpll
  Goto Tag Visibility8 : GotoTagVisibility  GotoTag=omega_grid_pll_pu
  Goto Tag Visibility9 : GotoTagVisibility  GotoTag=phase_grid_pll
  acquisitions : Subsystem
  current_ctrl : Subsystem
  data_to_worspace_module_1 : Subsystem
  grid_voltage_phase_lock_loops : Subsystem
  instantaneus_power : Subsystem
  interesting scopes : Subsystem
  power-meter mod1 : Scope  NumInputPorts=2
      settings: ActiveDisplayYMinimum=-23.563877806732968  ActiveDisplayYMaximum=-23.184007356049328  DataLoggingVariableName=ScopeData9
  space_vector : Subsystem
  udc_ctrl : Subsystem
  duvw : Outport
  AFE1_local_time_corr : Outport  Port=2
  m_data : Outport  Port=3
  tag scope: local_time=scoped, v_grid_ff_abc=scoped
  wires:
  current_ctrl/1(uabg) -> space_vector/1(uab_out)
  space_vector/1(duvw) -> duvw/1
  [ugd_abc_pu] -> grid_voltage_phase_lock_loops/1(ug_abc_pu)
  [udcd_pu_afe] -> udc_ctrl/1(udc_pu)
  [pwr_react_grid] -> power-meter mod1/2  "pwr_react_grid_mod1(kVAr)"
  [pwr_act_grid] -> power-meter mod1/1  "pwr_act_grid_mod1(kW)"
  local_time/1 -> [local_time]
  [ugd_abc_pu] -> [v_grid_ff_abc]
  data_to_worspace_module_1/1(m) -> m_data/1
  ug_abc_pu/1 -> acquisitions/1(ug_abc_pu)
  udc_pu/1 -> acquisitions/2(udc_pu)
  ig_abc_pu/1 -> acquisitions/3(ig_abc_pu)
  is_abc_pu/1 -> acquisitions/4(is_abc_pu)
  master_time/1 -> acquisitions/5(master_time)
  grid_phase/1 -> acquisitions/6(grid_phase)
  acquisitions/1(AFE1_local_time_corr) -> AFE1_local_time_corr/1
  udc_ctrl/1(i_xi_ref) -> current_ctrl/1(i_xi_ref)

== system afe_dqctrl_param/afe_dq_mod1/LCL_filter/threephase_vi_measures_stack ==
  Bus Creator : BusCreator  Inputs=6
  Current Sensor : fl_lib/Electrical/Electrical Sensors/Current Sensor
  Current Sensor1 : fl_lib/Electrical/Electrical Sensors/Current Sensor
  Current Sensor2 : fl_lib/Electrical/Electrical Sensors/Current Sensor
  Electrical Reference1 : fl_lib/Electrical/Electrical Elements/Electrical Reference
  Gain : Gain  Gain=1/3
  Gain1 : Gain  Gain=1/param.afe.hw.ubez
  Gain2 : Gain  Gain=1/param.afe.hw.ubez
  Gain3 : Gain  Gain=1/param.afe.hw.ubez
  Gain4 : Gain  Gain=1/param.afe.hw.ibez
  Gain5 : Gain  Gain=1/param.afe.hw.ibez
  Gain6 : Gain  Gain=1/param.afe.hw.ibez
  Selector : Selector  InputPortWidth=6  IndexOptions=Index vector (dialog)  Indices=[1 2 3]  OutputSizes=1
  Selector1 : Selector  InputPortWidth=6  IndexOptions=Index vector (dialog)  Indices=[4 5 6]  OutputSizes=1
  Sum : Sum  Inputs=+++
  Voltage Sensor : fl_lib/Electrical/Electrical Sensors/Voltage Sensor
  Voltage Sensor1 : fl_lib/Electrical/Electrical Sensors/Voltage Sensor
  Voltage Sensor2 : fl_lib/Electrical/Electrical Sensors/Voltage Sensor
  ia_afe : nesl_utility/PS-Simulink Converter  PhysicalDomain=network_engine_domain  SubClassName=ps_output  LeftPortType=input  RightPortType=output  PseudoPeriodic=off  Frequencies=[]  VectorFormat=1-D array  Unit=A  AffineConversion=off
  ib_afe : nesl_utility/PS-Simulink Converter  PhysicalDomain=network_engine_domain  SubClassName=ps_output  LeftPortType=input  RightPortType=output  PseudoPeriodic=off  Frequencies=[]  VectorFormat=1-D array  Unit=A  AffineConversion=off
  ic_afe : nesl_utility/PS-Simulink Converter  PhysicalDomain=network_engine_domain  SubClassName=ps_output  LeftPortType=input  RightPortType=output  PseudoPeriodic=off  Frequencies=[]  VectorFormat=1-D array  Unit=A  AffineConversion=off
  ua_afe : nesl_utility/PS-Simulink Converter  PhysicalDomain=network_engine_domain  SubClassName=ps_output  LeftPortType=input  RightPortType=output  PseudoPeriodic=off  Frequencies=[]  VectorFormat=1-D array  Unit=V  AffineConversion=off
  ub_afe : nesl_utility/PS-Simulink Converter  PhysicalDomain=network_engine_domain  SubClassName=ps_output  LeftPortType=input  RightPortType=output  PseudoPeriodic=off  Frequencies=[]  VectorFormat=1-D array  Unit=V  AffineConversion=off
  uc_afe : nesl_utility/PS-Simulink Converter  PhysicalDomain=network_engine_domain  SubClassName=ps_output  LeftPortType=input  RightPortType=output  PseudoPeriodic=off  Frequencies=[]  VectorFormat=1-D array  Unit=V  AffineConversion=off
  Ua : PMIOPort  Side=Left
  ua : PMIOPort  Port=2  Side=Right
  Ub : PMIOPort  Port=3  Side=Left
  ub : PMIOPort  Port=4  Side=Right
  Uc : PMIOPort  Port=5  Side=Left
  uc : PMIOPort  Port=6  Side=Right
  tag scope: is_abc_pu_mod1=global, iz_afe_pu_mod1=global, vs_abc_pu_mod1=global
  wires:
  Bus Creator/1 -> Selector/1, Selector1/1  "vi_data"
  Selector/1 -> [vs_abc_pu_mod1]
  ib_afe/1 -> Gain4/1  "ib_afe"
  ia_afe/1 -> Gain6/1  "ia_afe"
  ic_afe/1 -> Gain5/1  "ic_afe"
  ua_afe/1 -> Gain1/1  "ua_afe"
  ub_afe/1 -> Gain2/1  "ub_afe"
  uc_afe/1 -> Gain3/1  "uc_afe"
  Selector1/1 -> [is_abc_pu_mod1]
  Sum/1 -> Gain/1
  Gain/1 -> [iz_afe_pu_mod1]
  Gain1/1 -> Bus Creator/1  "ua_afe_pu"
  Gain2/1 -> Bus Creator/2  "ub_afe_pu"
  Gain3/1 -> Bus Creator/3  "uc_afe_pu"
  Gain6/1 -> Sum/1, Bus Creator/4  "ia_afe_pu"
  Gain4/1 -> Sum/2, Bus Creator/5  "ib_afe_pu"
  Gain5/1 -> Bus Creator/6, Sum/3  "ic_afe_pu"
  connections:
  Current Sensor1/LConn1 -- Ub/RConn1 -- Voltage Sensor1/LConn1
  Electrical Reference1/LConn1 -- Voltage Sensor/RConn2 -- Voltage Sensor2/RConn2 -- Voltage Sensor1/RConn2
  Voltage Sensor/RConn1 -- ua_afe/LConn1
  Current Sensor/RConn2 -- ua/RConn1
  Voltage Sensor1/RConn1 -- ub_afe/LConn1
  Voltage Sensor2/LConn1 -- Uc/RConn1 -- Current Sensor2/LConn1
  Current Sensor/LConn1 -- Ua/RConn1 -- Voltage Sensor/LConn1
  Current Sensor1/RConn2 -- ub/RConn1
  Voltage Sensor2/RConn1 -- uc_afe/LConn1
  ib_afe/LConn1 -- Current Sensor1/RConn1
  ia_afe/LConn1 -- Current Sensor/RConn1
  ic_afe/LConn1 -- Current Sensor2/RConn1
  Current Sensor2/RConn2 -- uc/RConn1

== system afe_dqctrl_param/afe_dq_mod1/LCL_filter/threephase_vi_measures_stack1 ==
  Bus Creator : BusCreator  Inputs=6
  Current Sensor : fl_lib/Electrical/Electrical Sensors/Current Sensor
  Current Sensor1 : fl_lib/Electrical/Electrical Sensors/Current Sensor
  Current Sensor2 : fl_lib/Electrical/Electrical Sensors/Current Sensor
  Electrical Reference1 : fl_lib/Electrical/Electrical Elements/Electrical Reference
  Gain1 : Gain  Gain=1/param.afe.hw.ubez
  Gain2 : Gain  Gain=1/param.afe.hw.ubez
  Gain3 : Gain  Gain=1/param.afe.hw.ubez
  Gain4 : Gain  Gain=1/param.afe.hw.ibez
  Gain5 : Gain  Gain=1/param.afe.hw.ibez
  Gain6 : Gain  Gain=1/param.afe.hw.ibez
  Selector : Selector  InputPortWidth=6  IndexOptions=Index vector (dialog)  Indices=[1 2 3]  OutputSizes=1
  Selector1 : Selector  InputPortWidth=6  IndexOptions=Index vector (dialog)  Indices=[4 5 6]  OutputSizes=1
  Voltage Sensor : fl_lib/Electrical/Electrical Sensors/Voltage Sensor
  Voltage Sensor1 : fl_lib/Electrical/Electrical Sensors/Voltage Sensor
  Voltage Sensor2 : fl_lib/Electrical/Electrical Sensors/Voltage Sensor
  ia_grid : nesl_utility/PS-Simulink Converter  PhysicalDomain=network_engine_domain  SubClassName=ps_output  LeftPortType=input  RightPortType=output  PseudoPeriodic=off  Frequencies=[]  VectorFormat=1-D array  Unit=A  AffineConversion=off
  ib_grid : nesl_utility/PS-Simulink Converter  PhysicalDomain=network_engine_domain  SubClassName=ps_output  LeftPortType=input  RightPortType=output  PseudoPeriodic=off  Frequencies=[]  VectorFormat=1-D array  Unit=A  AffineConversion=off
  ic_grid : nesl_utility/PS-Simulink Converter  PhysicalDomain=network_engine_domain  SubClassName=ps_output  LeftPortType=input  RightPortType=output  PseudoPeriodic=off  Frequencies=[]  VectorFormat=1-D array  Unit=A  AffineConversion=off
  ua_grid : nesl_utility/PS-Simulink Converter  PhysicalDomain=network_engine_domain  SubClassName=ps_output  LeftPortType=input  RightPortType=output  PseudoPeriodic=off  Frequencies=[]  VectorFormat=1-D array  Unit=V  AffineConversion=off
  ub_grid : nesl_utility/PS-Simulink Converter  PhysicalDomain=network_engine_domain  SubClassName=ps_output  LeftPortType=input  RightPortType=output  PseudoPeriodic=off  Frequencies=[]  VectorFormat=1-D array  Unit=V  AffineConversion=off
  uc_grid : nesl_utility/PS-Simulink Converter  PhysicalDomain=network_engine_domain  SubClassName=ps_output  LeftPortType=input  RightPortType=output  PseudoPeriodic=off  Frequencies=[]  VectorFormat=1-D array  Unit=V  AffineConversion=off
  Ua : PMIOPort  Side=Left
  ua : PMIOPort  Port=2  Side=Right
  Ub : PMIOPort  Port=3  Side=Left
  ub : PMIOPort  Port=4  Side=Right
  Uc : PMIOPort  Port=5  Side=Left
  uc : PMIOPort  Port=6  Side=Right
  tag scope: ig_abc_pu_mod1=global, ug_abc_pu_mod1=global
  wires:
  Selector1/1 -> [ig_abc_pu_mod1]
  uc_grid/1 -> Gain3/1
  ub_grid/1 -> Gain2/1
  ua_grid/1 -> Gain1/1
  ic_grid/1 -> Gain5/1
  ia_grid/1 -> Gain6/1
  ib_grid/1 -> Gain4/1
  Selector/1 -> [ug_abc_pu_mod1]
  Bus Creator/1 -> Selector1/1, Selector/1  "vi_data"
  Gain1/1 -> Bus Creator/1  "ua_grid_pu"
  Gain2/1 -> Bus Creator/2  "ub_grid_pu"
  Gain3/1 -> Bus Creator/3  "uc_grid_pu"
  Gain6/1 -> Bus Creator/4  "ia_grid_pu"
  Gain4/1 -> Bus Creator/5  "ib_grid_pu"
  Gain5/1 -> Bus Creator/6  "ic_grid_pu"
  connections:
  Current Sensor2/RConn2 -- uc/RConn1
  ic_grid/LConn1 -- Current Sensor2/RConn1
  ia_grid/LConn1 -- Current Sensor/RConn1
  ib_grid/LConn1 -- Current Sensor1/RConn1
  Voltage Sensor2/RConn1 -- uc_grid/LConn1
  Current Sensor1/RConn2 -- ub/RConn1
  Voltage Sensor/LConn1 -- Current Sensor/LConn1 -- Ua/RConn1
  Current Sensor2/LConn1 -- Voltage Sensor2/LConn1 -- Uc/RConn1
  Voltage Sensor1/RConn1 -- ub_grid/LConn1
  Current Sensor/RConn2 -- ua/RConn1
  Voltage Sensor/RConn1 -- ua_grid/LConn1
  Voltage Sensor1/RConn2 -- Voltage Sensor2/RConn2 -- Voltage Sensor/RConn2 -- Electrical Reference1/LConn1
  Voltage Sensor1/LConn1 -- Current Sensor1/LConn1 -- Ub/RConn1
